simulink model "SolarPowerInverter"  (R2025a)
settings: Solver=VariableStepAuto  StartTime=0.0  StopTime=1/60  RelTol=1e-4  AbsTol=1e-3  EnableMultiTasking=on
PreLoadFcn:
  | irradiance = 1000;
  | i_ac_ref = 20.05;
  | v_dc_ref = 342;
  | temperature = 20;
  | f_pwm = 10000;
  | L = 0.005;
  | C = 5000e-6;
  | ts = 1/f_pwm/10;
  | v_ac_nom = 110;
undefined symbols (not defined in the file or in its folder): DiscIntNeverNeededParam
libraries: ee_lib x18, fl_lib x12, nesl_utility x10
CloseFcn:
  | try,close(h1_SolarPowerInverter),end
  | clear h1_SolarPowerInverter
  | 
  | clear simlog_SolarPowerInverter
  | clear logsout_SolarPowerInverter
  | clear C L efficiency f_pwm iDC i_ac_ref irradiance powerDC powerLosses t tabulatedLosses temperature totalLosses ts vDC v_ac_nom v_dc_ref
Description:
  | Solar Power Inverter
settings Model: Creator=The MathWorks, Inc.  LastModifiedBy=The MathWorks, Inc.
settings SolverCC: AutoScaleAbsTol=off  MaxConsecutiveMinStep=50  AlgebraicLoopSolver=TrustRegion
settings DataIOCC: MaxDataPoints=210000  SaveFormat=Array  SaveOutput=off  SignalLogging=off  DSMLogging=off  SaveTime=off  ReturnWorkspaceOutputs=off  SignalLoggingName=logsout_SolarPowerInverter  OutputTimes=[0:0.005:60]
settings OptimizationCC: ReuseModelBlockBuffer=off  ExpressionDepthLimit=2147483647.0  LifeSpan=inf
settings DebuggingCC: UnderspecifiedInitializationDetection=Classic  MergeDetectMultiDrivingBlocksExec=none  FcnCallInpInsideContextMsg=warning  UnconnectedInputMsg=warning  UnconnectedOutputMsg=warning  UnconnectedLineMsg=warning  AllowSymbolicDim=off  StateNameClashWarn=warning  SFUnexpectedBacktrackingDiag=warning  SFNoUnconditionalDefaultTransitionDiag=warning  SFExecutionAtInitializationDiag=none  ArithmeticOperatorsInVariantConditions=warning
settings HardwareCC: ProdBitPerPointer=32.0  ProdBitPerSizeT=32.0  ProdBitPerPtrDiffT=32.0  ProdLargestAtomicFloat=None  ProdIntDivRoundTo=Undefined  ProdEndianess=Unspecified  ProdWordSize=32.0  ProdHWDeviceType=32-bit Generic
settings ModelReferenceCC: EnableRefExpFcnMdlSchedulingChecks=on  PropagateSignalLabelsOutOfModel=off
settings SFSimCC: SimUseLocalCustomCode=off  CustomCodeUndefinedFunction=UseInterfaceOnly
settings RTWCC: RTWUseLocalCustomCode=off  GPUComputeCapability=3.5  DLArmComputeVersion=19.05
settings CodeAppCC: StateflowObjectComments=on
settings GRTTargetCC: TargetLangStandard=C89/C90 (ANSI)  CombineOutputUpdateFcns=off  GRTInterface=on
settings ConfigComp: CovMetricSettings=dw  CovSaveCumulativeToWorkspaceVar=on  CovSaveSingleToWorkspaceVar=on  CovExternalEMLEnable=off  CovSFcnEnable=off
settings SimscapeCC: SimscapeLogType=local  SimscapeLogSimulationStatistics=on  SimscapeLogName=simlog_SolarPowerInverter  SimscapeLogLimitData=off  SimscapeLogDataHistory=210000.0

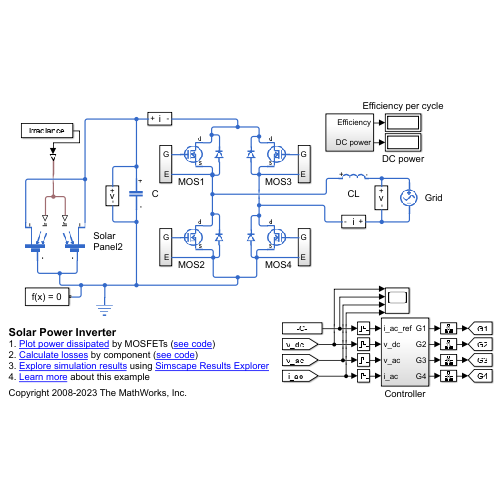
[thumbnail: Simulink's stored preview of the top-level diagram]
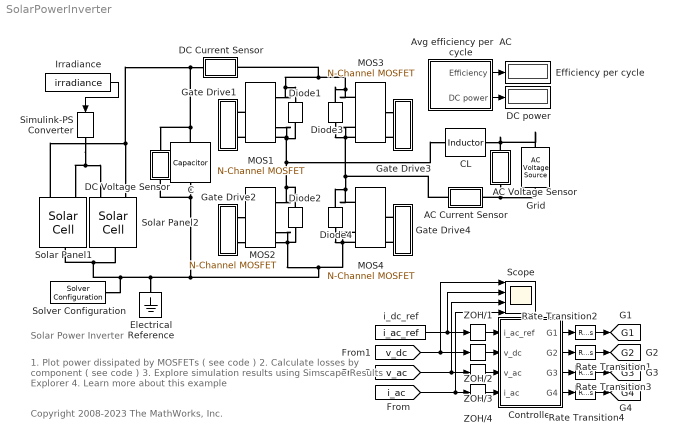
== system SolarPowerInverter ==
  note: Solar Power Inverter
  note: 1. Plot power dissipated by MOSFETs ( see code )
      | 2. Calculate losses by component ( see code )
      | 3. Explore simulation results using Simscape Results Explorer
      | 4. Learn more about this example
  note: Copyright 2008-2023 The MathWorks, Inc.
  AC Current Sensor : Subsystem
      mask Display: disp('i');
  AC Voltage Sensor : Subsystem
      mask Display: disp('v')
  Avg efficiency per  AC cycle : Subsystem
  C : fl_lib/Electrical/Electrical Elements/Capacitor  c=C F  r=1e-6 Ohm  g=0 1/Ohm  i_specify=off  i_priority=High  i=0 A  i_nominal_specify=off  i_nominal_value=1  i_nominal_unit=A  v_specify=off  v_priority=High  v=0 V  v_nominal_specify=off  v_nominal_value=1  v_nominal_unit=V  vc_specify=on  vc_priority=High  vc=v_dc_ref V  vc_nominal_specify=off  vc_nominal_value=1  vc_nominal_unit=V
  CL : fl_lib/Electrical/Electrical Elements/Inductor  l=L H  r=1e-3 Ohm  g=1e-9 1/Ohm  i_specify=off  i_priority=High  i=0 A  i_nominal_specify=off  i_nominal_value=1  i_nominal_unit=A  v_specify=off  v_priority=High  v=0 V  v_nominal_specify=off  v_nominal_value=1  v_nominal_unit=V  i_L_specify=on  i_L_priority=High  i_L=0 A  i_L_nominal_specify=off  i_L_nominal_value=1  i_L_nominal_unit=A
      settings: LogSimulationData=on
  Controller : Subsystem
  DC Current Sensor : Subsystem
      mask Display: disp('i')
  DC Voltage Sensor : Subsystem
      mask Display: disp('v');
  DC power : Display
  Diode{1..4} (4 alike) : ee_lib/Semiconductors & Converters/Diode  ModelType=ee.enum.diode.modelType.exponential  TableType=ee.enum.diode.tableType.IfMat  IfMat=[.07, .12, .19, 1.75, 4.24, 7.32, 11.2; .16, .3, .72, 2.14, 4.02, 6.35, 9.12] A  VfMat=[.9, 1.15, 1.25, 1.5, 1.75, 2.17, 2.6, 2.85; .58, .68, .75, 1.1, 1.38, 1.77, 2.27, 2.7] V  TjVec=[25, 125] degC  VfVec=[.5, .7, .9, 1.3, 1.7, 2.1, 2.5] V  IfVec=[.1, .2, .5, 1, 2, 4, 7, 10] A  IrMat=[1e-06, 2e-06, 5e-06, 1e-05, 2.5e-05, 5e-05, .0001; 2e-06, 5e-06, 1e-05, 4e-05, 8e-05, .0002, .0005] A  VrMat=[10, 100, 200, 250, 300, 325, 350; 10, 70, 160, 220, 270, 300, 320] V  VrVec=[10, 20, 40, 50, 70, 80, 100] V  IrVec=[1e-06, 2e-06, 5e-06, 1e-05, 2e-05, 5e-05, .0001] A  Vf=0.6 V  Ron=0.001 Ohm  Goff=1e-8 S  prmExp=1  I12=[ 0.137 5.45 ] A  V12=[ 0.6 0.7 ] V  RS=0.01 Ohm  Tmeas=25 degC  IS=1e-12 A  ec=1  I1=0.0137 A  V1=0.6 V  N_series=1  N_parallel=1  ZenerEnable=false  Rz=0.3 Ohm  BV=Inf V  C_param=1  CJ=50 pF  CJ0=50 pF  Vvec=[ 0.1 10 100 ] V  Cvec=[ 3.5 1 0.4 ] pF  VJ=1 V  Mgrad=0.5  FC=0.5  Q_param=ee.enum.diode.recoveryParam.off  iRM=-7.15 A  iF=4 A  didt=-750 A/us  trr_factor=3  trr=115 ns  Qrr=1500 s*uA  Vr=-600 V  Ls=150 nH  Erec=0.03 J  TT=50 ns  tau=100 ns  T_param=1  Tdevice=25 degC  I1_T2=0.245 A  V1_T2=0.5 V  IS_T2=1.25e-7 A  Tmeas2=125 degC  XTI_param=1  XTI=3  EG_param=1  EG=1.11 eV  dBVdT=0 V/K  enable_fault_input=simscape.enum.onoff.off  i_specify=off  i_priority=None  i=0 A  i_nominal_specify=off  i_nominal_value=1  i_nominal_unit=A  v_specify=off  v_priority=None  v=0 V  v_nominal_specify=off  v_nominal_value=1  v_nominal_unit=V  v_capacitor_specify=off  v_capacitor_priority=None  v_capacitor=0 V  v_capacitor_nominal_specify=off  v_capacitor_nominal_value=1  v_capacitor_nominal_unit=V  Qj_specify=off  Qj_priority=High  Qj=0 C  Qj_nominal_specify=off  Qj_nominal_value=1  Qj_nominal_unit=C  i_diode_specify=off  i_diode_priority=None  i_diode=0 A  i_diode_nominal_specify=off  i_diode_nominal_value=1  i_diode_nominal_unit=A  v_diode_specify=off  v_diode_priority=None  v_diode=0 V  v_diode_nominal_specify=off  v_diode_nominal_value=1  v_diode_nominal_unit=V  i_capacitor_specify=off  i_capacitor_priority=High  i_capacitor=0 A  i_capacitor_nominal_specify=off  i_capacitor_nominal_value=1  i_capacitor_nominal_unit=A  power_dissipated_specify=off  power_dissipated_priority=None  power_dissipated=0 W  power_dissipated_nominal_specify=off  power_dissipated_nominal_value=1  power_dissipated_nominal_unit=W  fidelity_level=ee.enum.diode.fidelity.includeChargeDyn  rec_loss_model=ee.enum.diode.reverseRecoveryModel.fixed  ErecVal=0 J  scaleWithIandV=true  ErecMat=zeros(2, 3) J  TjrecVec=[298.15, 398.15] K  IfrecVec=[.1, 1, 10] A  IrecVal=10 A  VrecVal=10 V  tFilter=1 / 1000 / 100 s  thermal_network_parameterization=ee.enum.thermalNetworkTopology.junctionCase  Rth=[0, 10] K/W  Rth_Cauer=[1, 3, 10] K/W  Rth_Foster=[4, 6] K/W  thermal_mass_parameterization=ee.enum.thermalNetwork.timeconstant  thermal_mass=[0, 1] J/K  thermal_mass_Cauer=[.1, .3, 1] J/K  thermal_mass_Foster=[1.5, 3] J/K  thermal_time_constant=[0, 10] s  thermal_time_constant_Cauer=[1, 3, 10] s  thermal_time_constant_Foster=[6, 18] s  thermal_mass_initial_temperatures=[25, 25] degC  thermal_mass_initial_temperatures_Cauer=[25, 25, 25] degC  junction_thermal_mass=0.01 J/K  Tvec_initial_Foster=[25, 25, 25, 25] degC  no_thermal_network=0  junction_temperature_specify=off  junction_temperature_priority=None  junction_temperature=25 degC  junction_temperature_nominal_specify=off  junction_temperature_nominal_value=1  junction_temperature_nominal_unit=degC
      settings: LogSimulationData=on
  Efficiency per cycle : Display
  Electrical Reference : fl_lib/Electrical/Electrical Elements/Electrical Reference
  Gate Drive1 : Subsystem
  Gate Drive2 : Subsystem
  Gate Drive3 : Subsystem
  Gate Drive4 : Subsystem
  Grid : fl_lib/Electrical/Electrical Sources/AC Voltage Source  amp=v_ac_nom*sqrt(2) V  shift=0 deg  frequency=60 Hz
  Irradiance : Constant  Value=irradiance
  MOS{1..4} (4 alike) : ee_lib/Semiconductors & Converters/N-Channel MOSFET  paramTerminal=ee.enum.mosfet.numberOfTerminals.three  parameterization=1  Beta=5 A/V^2  Rds=0.1 Ohm  Id=15 A  Vgs=10 V  Vth=1.7 V  Vth0=1.7 V  lam=0 1/V  gamma_vth=0.5 V^0.50000  phib=0.5 V  Vth1=1.9071 V  Vbs1=-1 V  Vth2=2.066 V  Vbs2=-2 V  Tmeas=25 degC  Vgs_vec=[-.5, 2, 3, 4, 5] V  Vds_vec=[0, 2, 4, 8, 12, 16, 20] V  Vbs_vec=[0, -4, -6, -12] V  T_vec=[25, 125] degC  Vth_vec=[.4, 1.2, 1.4, 1.45] V  Vth_mat=[.4, .35; 1.2, 1.15; 1.4, 1.35; 1.45, 1.4] V  Ids_mat=[0, 0, 0, 0, 0, 0, 0; 0, .003, .0038, .0043, .0046, .0048, .0049; 0, .0055, .008, .009, .0095, .01, .0101; 0, .0115, .016, .018, .019, .0195, .02; 0, .0152, .0225, .0265, .028, .0295, .03] A  Ids_mat0=[0, 0, 0, 0, 0, 0, 0; 0, .003, .0038, .0043, .0046, .0048, .0049; 0, .0055, .008, .009, .0095, .01, .0101; 0, .0115, .016, .018, .019, .0195, .02; 0, .0152, .0225, .0265, .028, .0295, .03] A  Ids_mat_3D=zeros(5, 7, 2) A  Ids_mat_3D0=zeros(5, 7, 2) A  IV_table_symmetry=ee.enum.mosfet.symmetricNIV.no  RS=0.01 Ohm  RD=0.01 Ohm  RB=0.001 Ohm  LeadRs=0 Ohm  LeadRd=0 Ohm  LeadRg=1e-3 Ohm  LeadRb=0 Ohm  LS=0 nH  LD=0 nH  LG=0 nH  LB=0 nH  C_param=1  C_GS=270 pF  C_GD=80 pF  C_GB=0 pF  C_DS=0 pF  C_iss=900 pF  C_rss=80 pF  C_oss=0 pF  C_iss_vec=[ 720 700 590 470 390 310 ] pF  C_rss_vec=[ 450 400 300 190 95 55 ] pF  C_oss_vec=[ 900 810 690 420 270 170 ] pF  C_GS_vec=[ 270 300 290 280 295 255 ] pF  C_GD_vec=[ 450 400 300 190 95 55 ] pF  C_GB_vec=[270, 300, 290, 280, 295, 255] pF  C_Vgs_vec=0 V  C_DS_vec=[ 450 410 390 230 175 115 ] pF  C_Vds_vec=[ 0.1 0.3 1 3 10 30 ] V  V_GS_for_cap_data=NaN V  charge_linearity_param=1  C_OX=200 pF  V_C_OX=-0.5 V  charge_linearity_param_vgb=ee.enum.mosfet.cgbLinearity.instantly  charge_linearity_param_with_vgb=ee.enum.mosfet.cgbLinearityWithSeparateCgb.instantly  Di_param=ee.enum.mosfet.diodeParam.exponential  IsDiode=0 A  Vbi=0.6 V  n=1  Cj0Diode=0 pF  TT=50e-9 s  Tmeas_dio=25 degC  TableTypeNoT=ee.enum.mosfet.tableType.IfMat  TableType=ee.enum.diode.tableType.IfMat  IfVec=[.07, .12, .19, 1.75, 4.24, 7.32, 11.2] A  IfMat=[.07, .12, .19, 1.75, 4.24, 7.32, 11.2; .16, .3, .72, 2.14, 4.02, 6.35, 9.12] A  VfVecV=[.9, 1.15, 1.25, 1.5, 1.75, 2.17, 2.6, 2.85] V  VfMatV=[.9, 1.15, 1.25, 1.5, 1.75, 2.17, 2.6, 2.85; .58, .68, .75, 1.1, 1.38, 1.77, 2.27, 2.7] V  TjVec=[25, 125] degC  VfVec=[.5, .7, .9, 1.3, 1.7, 2.1, 2.5] V  IfVecV=[.1, .2, .5, 1, 2, 4, 7, 10] A  diode_Goff=1e-12 1/Ohm  prmDatasheet=1  prmEquCoeff=1  dVth_dT=-6 mV/K  dVth0_dT=-6 mV/K  Rds_T2=0.037 Ohm  BEXDatasheet=-1.5  BEXEquCoeff=-1.5  etaisDatasheet=3  etaisEquCoeff=3  Tmeas2=125 degC  etaisTabulated=3  TdeviceDatasheet=25 degC  TdeviceEquCoeff=25 degC  TdeviceTabulated=25 degC  i_g_specify=off  i_g_priority=None  i_g=0 A  i_g_nominal_specify=off  i_g_nominal_value=1  i_g_nominal_unit=A  i_d_specify=off  i_d_priority=None  i_d=0 A  i_d_nominal_specify=off  i_d_nominal_value=1  i_d_nominal_unit=A  i_b_specify=off  i_b_priority=None  i_b=0 A  i_b_nominal_specify=off  i_b_nominal_value=1  i_b_nominal_unit=A  voltage_gs_specify=off  voltage_gs_priority=None  voltage_gs=0 V  voltage_gs_nominal_specify=off  voltage_gs_nominal_value=1  voltage_gs_nominal_unit=V  voltage_ds_specify=off  voltage_ds_priority=None  voltage_ds=0 V  voltage_ds_nominal_specify=off  voltage_ds_nominal_value=1  voltage_ds_nominal_unit=V  voltage_bs_specify=off  voltage_bs_priority=None  voltage_bs=0 V  voltage_bs_nominal_specify=off  voltage_bs_nominal_value=1  voltage_bs_nominal_unit=V  v_Cgs_specify=off  v_Cgs_priority=High  v_Cgs=0 V  v_Cgs_nominal_specify=off  v_Cgs_nominal_value=1  v_Cgs_nominal_unit=V  v_Cds_specify=off  v_Cds_priority=High  v_Cds=0 V  v_Cds_nominal_specify=off  v_Cds_nominal_value=1  v_Cds_nominal_unit=V  v_Cbs_specify=off  v_Cbs_priority=High  v_Cbs=0 V  v_Cbs_nominal_specify=off  v_Cbs_nominal_value=1  v_Cbs_nominal_unit=V  thermal_network_parameterization=ee.enum.thermalNetworkTopology.junctionCase  Rth=[0, 10] K/W  Rth_Cauer=[1, 3, 10] K/W  Rth_Foster=[4, 6] K/W  thermal_mass_parameterization=ee.enum.thermalNetwork.timeconstant  thermal_mass=[0, 1] J/K  thermal_mass_Cauer=[.1, .3, 1] J/K  thermal_mass_Foster=[1.5, 3] J/K  thermal_time_constant=[0, 10] s  thermal_time_constant_Cauer=[1, 3, 10] s  thermal_time_constant_Foster=[6, 18] s  thermal_mass_initial_temperatures=[25, 25] degC  thermal_mass_initial_temperatures_Cauer=[25, 25, 25] degC  Tvec_initial_Foster=[25, 25, 25, 25] degC  betaref=18 A/V^2  Vfbref=-1.1 V  gamma=3.5 V^(1/2)  phib2ref=1 V  thesatref=0.4 1/V  alpha=0  Vp=5e-2 V  thesrref=0 1/V  m=8  Tref=25 degC  Rsref=2e-3 Ohm  Rdref=0.17 Ohm  Rgref=8.4 Ohm  Rbref=2e-3 Ohm  Cox=1500 pF  Cgso=100 pF  Cgdo=14 pF  Isref=5.2e-13 A  Cj0=480 pF  Tprm=1  etabet=1.3  Stvfb=5e-4 V/K  Stphib=-8.5e-4 V/K  etasat=1.04  etasr=0.65  etar=0.95  etais=3  Tsim=25 degC  Ig_specify=off  Ig_priority=None  Ig=0 A  Ig_nominal_specify=off  Ig_nominal_value=1  Ig_nominal_unit=A  Ids_specify=off  Ids_priority=None  Ids=0 A  Ids_nominal_specify=off  Ids_nominal_value=1  Ids_nominal_unit=A  Ib_specify=off  Ib_priority=None  Ib=0 A  Ib_nominal_specify=off  Ib_nominal_value=1  Ib_nominal_unit=A  V_gs_specify=off  V_gs_priority=None  V_gs=0 V  V_gs_nominal_specify=off  V_gs_nominal_value=1  V_gs_nominal_unit=V  V_ds_specify=off  V_ds_priority=None  V_ds=0 V  V_ds_nominal_specify=off  V_ds_nominal_value=1  V_ds_nominal_unit=V  V_bs_specify=off  V_bs_priority=None  V_bs=0 V  V_bs_nominal_specify=off  V_bs_nominal_value=1  V_bs_nominal_unit=V  QGoverCox_specify=off  QGoverCox_priority=None  QGoverCox=0 V  QGoverCox_nominal_specify=off  QGoverCox_nominal_value=1  QGoverCox_nominal_unit=V  QDoverCox_specify=off  QDoverCox_priority=None  QDoverCox=0 V  QDoverCox_nominal_specify=off  QDoverCox_nominal_value=1  QDoverCox_nominal_unit=V  QBoverCox_specify=off  QBoverCox_priority=None  QBoverCox=0 V  QBoverCox_nominal_specify=off  QBoverCox_nominal_value=1  QBoverCox_nominal_unit=V  T0=[25, 25] degC  T0_Cauer=[25, 25, 25] degC
      settings: LogSimulationData=on
  Rate Transition{1..4} (4 alike) : RateTransition
  Scope : Scope  NumInputPorts=4
      settings: Title=DC voltage  ActiveDisplayYMinimum=0  ActiveDisplayYMaximum=400  DataLoggingMaxPoints=400000  DataLoggingVariableName=ScopeData4
  Simulink-PS Converter : nesl_utility/Simulink-PS Converter  PhysicalDomain=network_engine_domain  SubClassName=ps_input  LeftPortType=input  RightPortType=output  PseudoPeriodic=off  Frequencies=[]  NoiseDistribution=none  NoiseParameters=[]  Unit=1  AffineConversion=off  FilteringAndDerivatives=zero  SimscapeFilterOrder=1  InputFilterTimeConstant=0.001  UdotUserProvided=1
  Solar Panel1 : ee_lib/Sources/Solar Cell  prm=3  Isc=3.8 A  Voc=0.586 V  Is=3.15e-07 A  Is2=0 A  Iph=3.80 A  Ir0=1000 W/m^2  ec=1.4  N2=2  Rs=0.0042 Ohm  Rp=10.1 Ohm  N_series=700  N_parallel=1  TIPH1=0.000805 1/K  EG=1.14 eV  TXIS1=3.38  TXIS2=3  TRS1=0  TRP1=0  Tmeas=25 degC  TFIXED=temperature degC  thermal_mass=100 J/K  initial_temperature=25 degC
  Solar Panel2 : ee_lib/Sources/Solar Cell  prm=3  Isc=3.8 A  Voc=0.586 V  Is=3.15e-07 A  Is2=0 A  Iph=3.80 A  Ir0=1000 W/m^2  ec=1.4  N2=2  Rs=0.0042 Ohm  Rp=10.1 Ohm  N_series=700  N_parallel=1  TIPH1=0.000805 1/K  EG=1.14 eV  TXIS1=3.38  TXIS2=3  TRS1=0  TRP1=0  Tmeas=25 degC  TFIXED=temperature degC  thermal_mass=100 J/K  initial_temperature=25 degC
  Solver Configuration : nesl_utility/Solver Configuration  PhysicalDomain=network_engine_domain  SubClassName=solver  LeftPortType=input  RightPortType=generic  Tones=[]  Harmonics=[]  SimulateNoise=off  Profile=off  UseLocalSampling=off  EnableSwitchedLinearOptims=on  FrequencyDomain=off  UseCCode=off  RelTol=0.001  AbsTol=1e-06  MinStep=1e-09  ToWorkspace=off  RevertToSquareIcSolve=off  NumHomotopyIterations=100  PhasorMode=off  PhasorModeNumHarmonics=1  ConsistencySolver=NEWTON_FTOL  IndexReductionMethod=DerivativeReplacement  DoDC=off  ResidualTolerance=1e-9  ConsistencyTolSource=GLOBAL  ConsistencyAbsTol=0.001  ConsistencyRelTol=0.001  ConsistencyTolFactor=0.001  UseLocalSolver=off  LocalSolverChoice=NE_TRAPEZOIDAL_ADVANCER  ResolveIndetEquations=on  FunctionEvalNumThread=1  LocalSolverSampleTime=1e-7  DoFixedCost=off  MaxNonlinIter=10  MaxModeIter=2  ComputeImpulses=off  ImpulseIterations=1  LinearAlgebra=auto  LinearAlgebraNumThread=0  EquationFormulation=NE_TIME_EF  DelaysMemoryBudget=1024  AutomaticFiltering=on  FilteringTimeConstant=0.001  PartitionStorageMethod=AS_NEEDED  PartitionMemoryBudget=1024  PartitionMethod=FAST  MultibodyUseLocalSolver=off  MultibodyLocalSolverChoice=ODE1  MultibodyLocalSolverSampleTime=0.001
  ZOH/{1..4} (4 alike) : ZeroOrderHold  SampleTime=ts
  i_dc_ref : Constant  Value=i_ac_ref
  tag scope: G1=global, G2=global, G3=global, G4=global
  wires:
  Irradiance/1 -> Simulink-PS Converter/1
  ZOH/3/1 -> Controller/3(v_ac)
  ZOH/4/1 -> Controller/4(i_ac)
  Controller/1(G1) -> Rate Transition2/1
  Rate Transition2/1 -> [G1]
  Controller/2(G2) -> Rate Transition1/1
  Rate Transition1/1 -> [G2]
  Controller/3(G3) -> Rate Transition3/1
  Rate Transition3/1 -> [G3]
  Controller/4(G4) -> Rate Transition4/1
  Rate Transition4/1 -> [G4]
  [v_dc] -> ZOH/2/1, Scope/1
  [v_ac] -> Scope/3, ZOH/3/1
  [i_ac] -> Scope/4, ZOH/4/1
  Avg efficiency per  AC cycle/1(Efficiency) -> Efficiency per cycle/1
  Avg efficiency per  AC cycle/2(DC power) -> DC power/1
  ZOH/2/1 -> Controller/2(v_dc)
  ZOH/1/1 -> Controller/1(i_ac_ref)
  i_dc_ref/1 -> ZOH/1/1, Scope/2
  connections:
  Simulink-PS Converter/RConn1 -- Solar Panel2/LConn1 -- Solar Panel1/LConn1
  Solar Panel1/LConn2 -- DC Voltage Sensor/RConn1 -- C/LConn1 -- DC Current Sensor/RConn1 -- Solar Panel2/LConn2
  Diode4/LConn1 -- Gate Drive4/RConn2 -- MOS4/RConn2 -- Electrical Reference/LConn1 -- Solver Configuration/RConn1 -- Solar Panel1/RConn1 -- Solar Panel2/RConn1 -- DC Voltage Sensor/LConn1 -- C/RConn1 -- Gate Drive2/RConn2 -- Diode2/LConn1 -- MOS2/RConn2
  Grid/LConn1 -- CL/RConn1 -- AC Voltage Sensor/RConn1
  AC Voltage Sensor/LConn1 -- Grid/RConn1 -- AC Current Sensor/RConn1
  MOS1/RConn2 -- Gate Drive1/RConn2 -- MOS2/RConn1 -- Diode2/RConn1 -- CL/LConn1 -- Diode1/LConn1
  AC Current Sensor/LConn1 -- Diode4/RConn1 -- MOS4/RConn1 -- Diode3/LConn1 -- Gate Drive3/RConn2 -- MOS3/RConn2
  MOS1/LConn1 -- Gate Drive1/RConn1
  Gate Drive2/RConn1 -- MOS2/LConn1
  MOS3/LConn1 -- Gate Drive3/RConn1
  Gate Drive4/RConn1 -- MOS4/LConn1
  MOS1/RConn1 -- Diode3/RConn1 -- MOS3/RConn1 -- DC Current Sensor/LConn1 -- Diode1/RConn1

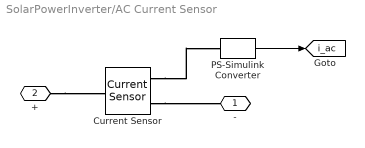
== system SolarPowerInverter/AC Current Sensor ==
  Current Sensor : fl_lib/Electrical/Electrical Sensors/Current Sensor
  PS-Simulink Converter : nesl_utility/PS-Simulink Converter  PhysicalDomain=network_engine_domain  SubClassName=ps_output  LeftPortType=input  RightPortType=output  PseudoPeriodic=off  Frequencies=[]  VectorFormat=1-D array  Unit=1  AffineConversion=off
  - : PMIOPort  Side=Left
  + : PMIOPort  Port=2  Side=Right
  tag scope: i_ac=global
  wires:
  PS-Simulink Converter/1 -> [i_ac]
  connections:
  Current Sensor/RConn1 -- PS-Simulink Converter/LConn1
  +/RConn1 -- Current Sensor/LConn1
  Current Sensor/RConn2 -- -/RConn1

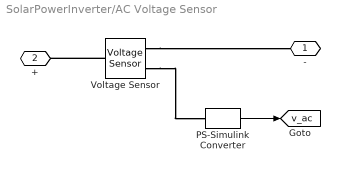
== system SolarPowerInverter/AC Voltage Sensor ==
  PS-Simulink Converter : nesl_utility/PS-Simulink Converter  PhysicalDomain=network_engine_domain  SubClassName=ps_output  LeftPortType=input  RightPortType=output  PseudoPeriodic=off  Frequencies=[]  VectorFormat=1-D array  Unit=1  AffineConversion=off
  Voltage Sensor : fl_lib/Electrical/Electrical Sensors/Voltage Sensor
  - : PMIOPort  Side=Left
  + : PMIOPort  Port=2  Side=Right
  tag scope: v_ac=global
  wires:
  PS-Simulink Converter/1 -> [v_ac]
  connections:
  Voltage Sensor/RConn2 -- -/RConn1
  Voltage Sensor/RConn1 -- PS-Simulink Converter/LConn1
  Voltage Sensor/LConn1 -- +/RConn1

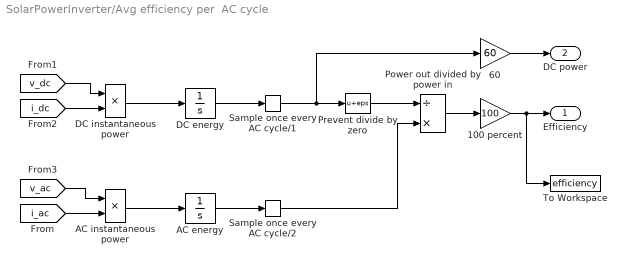
== system SolarPowerInverter/Avg efficiency per  AC cycle ==
  100 percent : Gain  Gain=100  SaturateOnIntegerOverflow=on  OutDataTypeStr=Inherit: Same as input  ParamDataTypeStr=Inherit: Same as input
  60 : Gain  Gain=60  SaturateOnIntegerOverflow=on  OutDataTypeStr=Inherit: Same as input  ParamDataTypeStr=Inherit: Same as input
  AC energy : Integrator
  AC instantaneous power : Product  InputSameDT=on  SaturateOnIntegerOverflow=on  OutDataTypeStr=Inherit: Same as first input
  DC energy : Integrator
  DC instantaneous power : Product  InputSameDT=on  SaturateOnIntegerOverflow=on  OutDataTypeStr=Inherit: Same as first input
  Power out divided by power in : Product  Inputs=/*  InputSameDT=on  SaturateOnIntegerOverflow=on  OutDataTypeStr=Inherit: Same as first input
  Prevent divide by zero : Bias  Bias=eps  SaturateOnIntegerOverflow=off
  Sample once every AC cycle/1 : ZeroOrderHold  SampleTime=1/60
  Sample once every AC cycle/2 : ZeroOrderHold  SampleTime=1/60
  To Workspace : ToWorkspace  VariableName=efficiency  SaveFormat=Structure  SampleTime=-1
      settings: MaxDataPoints=1
  Efficiency : Outport  VectorParamsAs1DForOutWhenUnconnected=off
  DC power : Outport  Port=2  VectorParamsAs1DForOutWhenUnconnected=off
  wires:
  [v_dc] -> DC instantaneous power/1
  [i_dc] -> DC instantaneous power/2
  [i_ac] -> AC instantaneous power/2
  [v_ac] -> AC instantaneous power/1
  DC instantaneous power/1 -> DC energy/1
  AC instantaneous power/1 -> AC energy/1
  AC energy/1 -> Sample once every AC cycle/2/1
  Power out divided by power in/1 -> 100 percent/1
  100 percent/1 -> To Workspace/1, Efficiency/1
  Sample once every AC cycle/1/1 -> Prevent divide by zero/1, 60/1
  Sample once every AC cycle/2/1 -> Power out divided by power in/2
  DC energy/1 -> Sample once every AC cycle/1/1
  60/1 -> DC power/1
  Prevent divide by zero/1 -> Power out divided by power in/1

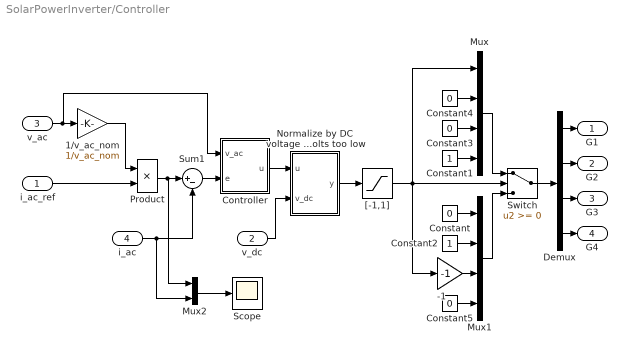
== system SolarPowerInverter/Controller ==
  i_ac_ref : Inport
  v_dc : Inport  Port=2
  v_ac : Inport  Port=3
  i_ac : Inport  Port=4
  -1 : Gain  Gain=-1  SaturateOnIntegerOverflow=on  OutDataTypeStr=Inherit: Same as input  ParamDataTypeStr=Inherit: Same as input
  1/v_ac_nom : Gain  Gain=1/v_ac_nom  SaturateOnIntegerOverflow=on  OutDataTypeStr=Inherit: Same as input  ParamDataTypeStr=Inherit: Same as input
  Constant{,3..5} (4 alike) : Constant  Value=0
  Constant1 : Constant
  Constant2 : Constant
  Controller : Subsystem
  Demux : Demux
  Mux : Mux
  Mux1 : Mux
  Mux2 : Mux  Inputs=2
  Normalize by DC voltage and disable if DC volts too low : Subsystem
  Product : Product  InputSameDT=on  SaturateOnIntegerOverflow=on  OutDataTypeStr=Inherit: Same as first input
  Scope : Scope
      settings: Title=Demanded and measured currents  ActiveDisplayYMinimum=-30  ActiveDisplayYMaximum=30
  Sum1 : Sum  Inputs=|+-  InputSameDT=on  SaturateOnIntegerOverflow=on  OutDataTypeStr=Inherit: Same as first input
  Switch : Switch  SaturateOnIntegerOverflow=off
  "[-1,1]" : Saturate  UpperLimit=1  LowerLimit=-1
  G1 : Outport  VectorParamsAs1DForOutWhenUnconnected=off
  G2 : Outport  Port=2  VectorParamsAs1DForOutWhenUnconnected=off
  G3 : Outport  Port=3  VectorParamsAs1DForOutWhenUnconnected=off
  G4 : Outport  Port=4  VectorParamsAs1DForOutWhenUnconnected=off
  wires:
  v_ac/1 -> Controller/1(v_ac), 1/v_ac_nom/1
  1/v_ac_nom/1 -> Product/1
  Product/1 -> Sum1/1, Mux2/1
  i_ac/1 -> Sum1/2, Mux2/2
  Switch/1 -> Demux/1
  Demux/1 -> G1/1
  Demux/2 -> G2/1
  Demux/3 -> G3/1
  Demux/4 -> G4/1
  Mux/1 -> Switch/1
  Constant/1 -> Mux1/1
  Mux1/1 -> Switch/3
  Constant1/1 -> Mux/4
  Constant3/1 -> Mux/3
  Constant4/1 -> Mux/2
  Constant5/1 -> Mux1/4
  -1/1 -> Mux1/3
  Constant2/1 -> Mux1/2
  "[-1,1]"/1 -> -1/1, Mux/1, Switch/2
  i_ac_ref/1 -> Product/2
  Mux2/1 -> Scope/1
  v_dc/1 -> Normalize by DC voltage and disable if DC volts too low/2(v_dc)
  Sum1/1 -> Controller/2(e)
  Controller/1(u) -> Normalize by DC voltage and disable if DC volts too low/1(u)
  Normalize by DC voltage and disable if DC volts too low/1(y) -> "[-1,1]"/1

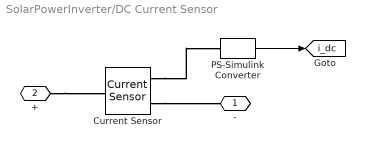
== system SolarPowerInverter/DC Current Sensor ==
  Current Sensor : fl_lib/Electrical/Electrical Sensors/Current Sensor
      settings: LogSimulationData=on
  PS-Simulink Converter : nesl_utility/PS-Simulink Converter  PhysicalDomain=network_engine_domain  SubClassName=ps_output  LeftPortType=input  RightPortType=output  PseudoPeriodic=off  Frequencies=[]  VectorFormat=1-D array  Unit=1  AffineConversion=off
  - : PMIOPort  Side=Left
  + : PMIOPort  Port=2  Side=Right
  tag scope: i_dc=global
  wires:
  PS-Simulink Converter/1 -> [i_dc]
  connections:
  Current Sensor/RConn2 -- -/RConn1
  +/RConn1 -- Current Sensor/LConn1
  Current Sensor/RConn1 -- PS-Simulink Converter/LConn1

== system SolarPowerInverter/DC Voltage Sensor ==
  PS-Simulink Converter : nesl_utility/PS-Simulink Converter  PhysicalDomain=network_engine_domain  SubClassName=ps_output  LeftPortType=input  RightPortType=output  PseudoPeriodic=off  Frequencies=[]  VectorFormat=1-D array  Unit=1  AffineConversion=off
  Voltage Sensor : fl_lib/Electrical/Electrical Sensors/Voltage Sensor
      settings: LogSimulationData=on
  - : PMIOPort  Side=Left
  + : PMIOPort  Port=2  Side=Right
  tag scope: v_dc=global
  wires:
  PS-Simulink Converter/1 -> [v_dc]
  connections:
  Voltage Sensor/LConn1 -- +/RConn1
  Voltage Sensor/RConn1 -- PS-Simulink Converter/LConn1
  Voltage Sensor/RConn2 -- -/RConn1

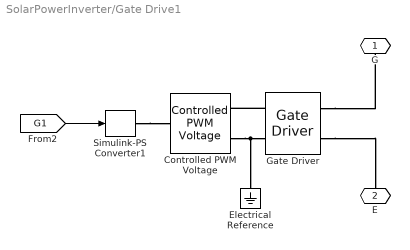
== system SolarPowerInverter/Gate Drive1 ==
  Controlled PWM Voltage : ee_lib/Integrated Circuits/Controlled PWM Voltage  F=f_pwm Hz  TD=0 s  pulse_width_offset=0 s  pulse_min=0 s  pwm_or_av=1  event_type=1  sample_time=1/f_pwm/100 s  Vmin=0 V  Vmax=5 V  Vm=5 V  u_min=0  u_max=1
      settings: InternalSimscapePortConfiguration="{\"Bottom\":[],\"Left\":[{\"id\":\"u\",\"label\":\"u\",\"type\":\"input\"}],\"Right\":[{\"id\":\"p2\",\"label\":\"PWM\",\"type\":\"foundation.electrical.electrical\"},{\"id\":\"n2\",\"label\":\"REF\",\"type\":\"foundation.electrical.electrical\"}],\"Top\":[]}"
  Electrical Reference : fl_lib/Electrical/Electrical Elements/Electrical Reference
  Gate Driver : ee_lib/Semiconductors & Converters/Gate Driver  port_option=ee.enum.controlport.elec  uHigh=3 V  uLow=2 V  uHighValue=0.7  uLowValue=0.3  vHigh=10 V  vLow=0 V  tHigh=200 ns  tLow=0 ns  parameterization=1  rHigh=10 Ohm  rLow=2 Ohm  tRise=20 ns  tFall=20 ns  cLoad=10 nF  ZonTime_specify=off  ZonTime_priority=None  ZonTime=0 s  ZoffTime_specify=off  ZoffTime_priority=None  ZoffTime=0 s
  Simulink-PS Converter1 : nesl_utility/Simulink-PS Converter  PhysicalDomain=network_engine_domain  SubClassName=ps_input  LeftPortType=input  RightPortType=output  PseudoPeriodic=off  Frequencies=[]  NoiseDistribution=none  NoiseParameters=[]  Unit=1  AffineConversion=off  FilteringAndDerivatives=zero  SimscapeFilterOrder=1  InputFilterTimeConstant=0.001  UdotUserProvided=1
  G : PMIOPort  Side=Right
  E : PMIOPort  Port=2  Side=Right
  wires:
  [G1] -> Simulink-PS Converter1/1
  connections:
  Simulink-PS Converter1/RConn1 -- Controlled PWM Voltage/LConn1
  Gate Driver/LConn1 -- Controlled PWM Voltage/RConn1
  Controlled PWM Voltage/RConn2 -- Electrical Reference/LConn1 -- Gate Driver/LConn2
  Gate Driver/RConn1 -- G/RConn1
  Gate Driver/RConn2 -- E/RConn1

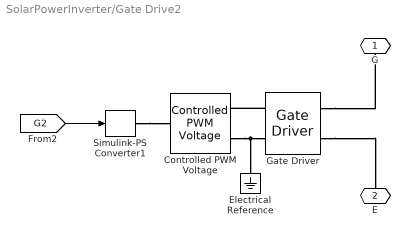
== system SolarPowerInverter/Gate Drive2 ==
  Controlled PWM Voltage : ee_lib/Integrated Circuits/Controlled PWM Voltage  F=f_pwm Hz  TD=0 s  pulse_width_offset=0 s  pulse_min=0 s  pwm_or_av=1  event_type=1  sample_time=1/f_pwm/100 s  Vmin=0 V  Vmax=5 V  Vm=5 V  u_min=0  u_max=1
      settings: InternalSimscapePortConfiguration="{\"Bottom\":[],\"Left\":[{\"id\":\"u\",\"label\":\"u\",\"type\":\"input\"}],\"Right\":[{\"id\":\"p2\",\"label\":\"PWM\",\"type\":\"foundation.electrical.electrical\"},{\"id\":\"n2\",\"label\":\"REF\",\"type\":\"foundation.electrical.electrical\"}],\"Top\":[]}"
  Electrical Reference : fl_lib/Electrical/Electrical Elements/Electrical Reference
  Gate Driver : ee_lib/Semiconductors & Converters/Gate Driver  port_option=ee.enum.controlport.elec  uHigh=3 V  uLow=2 V  uHighValue=0.7  uLowValue=0.3  vHigh=10 V  vLow=0 V  tHigh=200 ns  tLow=0 ns  parameterization=1  rHigh=10 Ohm  rLow=2 Ohm  tRise=20 ns  tFall=20 ns  cLoad=10 nF  ZonTime_specify=off  ZonTime_priority=None  ZonTime=0 s  ZoffTime_specify=off  ZoffTime_priority=None  ZoffTime=0 s
  Simulink-PS Converter1 : nesl_utility/Simulink-PS Converter  PhysicalDomain=network_engine_domain  SubClassName=ps_input  LeftPortType=input  RightPortType=output  PseudoPeriodic=off  Frequencies=[]  NoiseDistribution=none  NoiseParameters=[]  Unit=1  AffineConversion=off  FilteringAndDerivatives=zero  SimscapeFilterOrder=1  InputFilterTimeConstant=0.001  UdotUserProvided=1
  G : PMIOPort  Side=Right
  E : PMIOPort  Port=2  Side=Right
  wires:
  [G2] -> Simulink-PS Converter1/1
  connections:
  Gate Driver/RConn2 -- E/RConn1
  Gate Driver/RConn1 -- G/RConn1
  Controlled PWM Voltage/RConn2 -- Electrical Reference/LConn1 -- Gate Driver/LConn2
  Gate Driver/LConn1 -- Controlled PWM Voltage/RConn1
  Simulink-PS Converter1/RConn1 -- Controlled PWM Voltage/LConn1

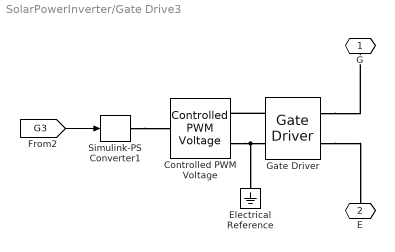
== system SolarPowerInverter/Gate Drive3 ==
  Controlled PWM Voltage : ee_lib/Integrated Circuits/Controlled PWM Voltage  F=f_pwm Hz  TD=0 s  pulse_width_offset=0 s  pulse_min=0 s  pwm_or_av=1  event_type=1  sample_time=1/f_pwm/100 s  Vmin=0 V  Vmax=5 V  Vm=5 V  u_min=0  u_max=1
      settings: InternalSimscapePortConfiguration="{\"Bottom\":[],\"Left\":[{\"id\":\"u\",\"label\":\"u\",\"type\":\"input\"}],\"Right\":[{\"id\":\"p2\",\"label\":\"PWM\",\"type\":\"foundation.electrical.electrical\"},{\"id\":\"n2\",\"label\":\"REF\",\"type\":\"foundation.electrical.electrical\"}],\"Top\":[]}"
  Electrical Reference : fl_lib/Electrical/Electrical Elements/Electrical Reference
  Gate Driver : ee_lib/Semiconductors & Converters/Gate Driver  port_option=ee.enum.controlport.elec  uHigh=3 V  uLow=2 V  uHighValue=0.7  uLowValue=0.3  vHigh=10 V  vLow=0 V  tHigh=200 ns  tLow=0 ns  parameterization=1  rHigh=10 Ohm  rLow=2 Ohm  tRise=20 ns  tFall=20 ns  cLoad=10 nF  ZonTime_specify=off  ZonTime_priority=None  ZonTime=0 s  ZoffTime_specify=off  ZoffTime_priority=None  ZoffTime=0 s
  Simulink-PS Converter1 : nesl_utility/Simulink-PS Converter  PhysicalDomain=network_engine_domain  SubClassName=ps_input  LeftPortType=input  RightPortType=output  PseudoPeriodic=off  Frequencies=[]  NoiseDistribution=none  NoiseParameters=[]  Unit=1  AffineConversion=off  FilteringAndDerivatives=zero  SimscapeFilterOrder=1  InputFilterTimeConstant=0.001  UdotUserProvided=1
  G : PMIOPort  Side=Right
  E : PMIOPort  Port=2  Side=Right
  wires:
  [G3] -> Simulink-PS Converter1/1
  connections:
  Gate Driver/LConn1 -- Controlled PWM Voltage/RConn1
  Simulink-PS Converter1/RConn1 -- Controlled PWM Voltage/LConn1
  Controlled PWM Voltage/RConn2 -- Electrical Reference/LConn1 -- Gate Driver/LConn2
  Gate Driver/RConn1 -- G/RConn1
  Gate Driver/RConn2 -- E/RConn1

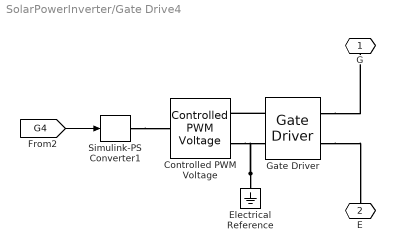
== system SolarPowerInverter/Gate Drive4 ==
  Controlled PWM Voltage : ee_lib/Integrated Circuits/Controlled PWM Voltage  F=f_pwm Hz  TD=0 s  pulse_width_offset=0 s  pulse_min=0 s  pwm_or_av=1  event_type=1  sample_time=1/f_pwm/100 s  Vmin=0 V  Vmax=5 V  Vm=5 V  u_min=0  u_max=1
      settings: InternalSimscapePortConfiguration="{\"Bottom\":[],\"Left\":[{\"id\":\"u\",\"label\":\"u\",\"type\":\"input\"}],\"Right\":[{\"id\":\"p2\",\"label\":\"PWM\",\"type\":\"foundation.electrical.electrical\"},{\"id\":\"n2\",\"label\":\"REF\",\"type\":\"foundation.electrical.electrical\"}],\"Top\":[]}"
  Electrical Reference : fl_lib/Electrical/Electrical Elements/Electrical Reference
  Gate Driver : ee_lib/Semiconductors & Converters/Gate Driver  port_option=ee.enum.controlport.elec  uHigh=3 V  uLow=2 V  uHighValue=0.7  uLowValue=0.3  vHigh=10 V  vLow=0 V  tHigh=200 ns  tLow=0 ns  parameterization=1  rHigh=10 Ohm  rLow=2 Ohm  tRise=20 ns  tFall=20 ns  cLoad=10 nF  ZonTime_specify=off  ZonTime_priority=None  ZonTime=0 s  ZoffTime_specify=off  ZoffTime_priority=None  ZoffTime=0 s
  Simulink-PS Converter1 : nesl_utility/Simulink-PS Converter  PhysicalDomain=network_engine_domain  SubClassName=ps_input  LeftPortType=input  RightPortType=output  PseudoPeriodic=off  Frequencies=[]  NoiseDistribution=none  NoiseParameters=[]  Unit=1  AffineConversion=off  FilteringAndDerivatives=zero  SimscapeFilterOrder=1  InputFilterTimeConstant=0.001  UdotUserProvided=1
  G : PMIOPort  Side=Right
  E : PMIOPort  Port=2  Side=Right
  wires:
  [G4] -> Simulink-PS Converter1/1
  connections:
  Gate Driver/RConn2 -- E/RConn1
  Gate Driver/RConn1 -- G/RConn1
  Electrical Reference/LConn1 -- Controlled PWM Voltage/RConn2 -- Gate Driver/LConn2
  Simulink-PS Converter1/RConn1 -- Controlled PWM Voltage/LConn1
  Gate Driver/LConn1 -- Controlled PWM Voltage/RConn1

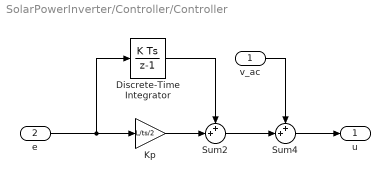
== system SolarPowerInverter/Controller/Controller ==
  v_ac : Inport
  e : Inport  Port=2
  Discrete-Time Integrator : DiscreteIntegrator  gainval=1000*L/ts  InitialCondition=15  SampleTime=ts  ICPrevOutput=DiscIntNeverNeededParam  ICPrevScaledInput=DiscIntNeverNeededParam
  Kp : Gain  Gain=L/ts/2  SaturateOnIntegerOverflow=on  OutDataTypeStr=Inherit: Same as input  ParamDataTypeStr=Inherit: Same as input
  Sum2 : Sum  Inputs=++|  InputSameDT=on  SaturateOnIntegerOverflow=on  OutDataTypeStr=Inherit: Same as first input
  Sum4 : Sum  Inputs=++|  InputSameDT=on  SaturateOnIntegerOverflow=on  OutDataTypeStr=Inherit: Same as first input
  u : Outport  VectorParamsAs1DForOutWhenUnconnected=off
  wires:
  e/1 -> Kp/1, Discrete-Time Integrator/1
  Kp/1 -> Sum2/2
  v_ac/1 -> Sum4/1
  Sum2/1 -> Sum4/2
  Sum4/1 -> u/1
  Discrete-Time Integrator/1 -> Sum2/1

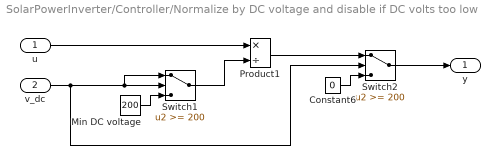
== system SolarPowerInverter/Controller/Normalize by DC voltage and disable if DC volts too low ==
  u : Inport
  v_dc : Inport  Port=2
  Constant6 : Constant  Value=0
  Min DC voltage : Constant  Value=200
  Product1 : Product  Inputs=*/  InputSameDT=on  SaturateOnIntegerOverflow=on  OutDataTypeStr=Inherit: Same as first input
  Switch1 : Switch  Threshold=200  SaturateOnIntegerOverflow=off
  Switch2 : Switch  Threshold=200  SaturateOnIntegerOverflow=off
  y : Outport  VectorParamsAs1DForOutWhenUnconnected=off
  wires:
  Min DC voltage/1 -> Switch1/3
  Constant6/1 -> Switch2/3
  Switch1/1 -> Product1/2
  Switch2/1 -> y/1
  v_dc/1 -> Switch2/2, Switch1/1, Switch1/2
  u/1 -> Product1/1
  Product1/1 -> Switch2/1
